simulink model "hdlcoder_led_blinking"  (R2026a)
settings: Solver=FixedStepDiscrete  StopTime=1
InitFcn:
  | Ts = 1e-3;
libraries: simulink x2, hdlsllib x2
settings Model: Creator=The MathWorks, Inc.  LastModifiedBy=The MathWorks, Inc.
settings OptimizationCC: ConditionallyExecuteInputs=off
settings DebuggingCC: AlgebraicLoopMsg=error  UnderspecifiedInitializationDetection=Classic  SingleTaskRateTransMsg=error  ParameterPrecisionLossMsg=none
settings HardwareCC: ProdHWDeviceType=ASIC/FPGA->ASIC/FPGA  ProdEqTarget=off

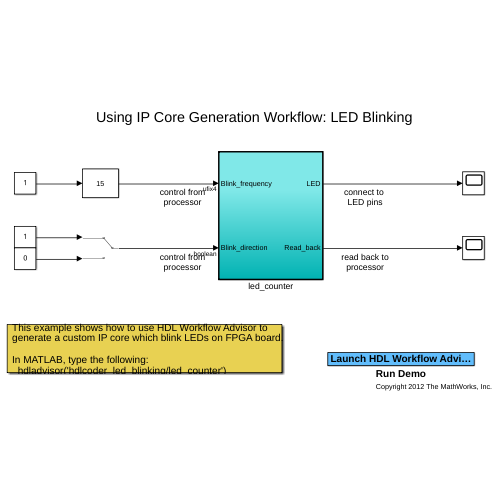
[thumbnail: Simulink's stored preview of the top-level diagram]
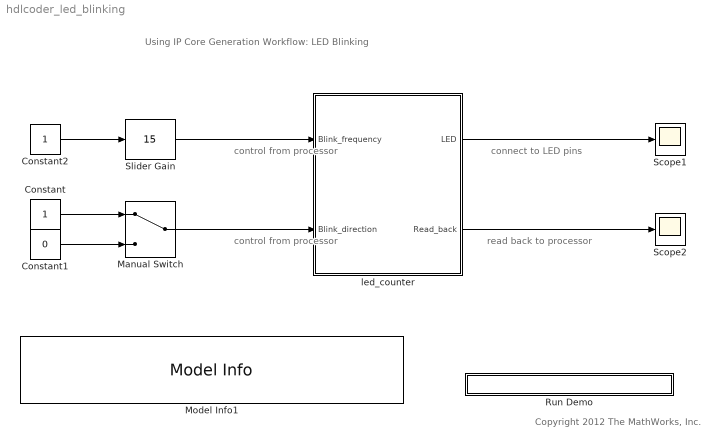
== system hdlcoder_led_blinking ==
  note: control from
      | processor
  note: Copyright 2012 The MathWorks, Inc.
  note: Using IP Core Generation Workflow: LED Blinking
  note: control from
      | processor
  note: connect to
      | LED pins
  note: read back to
      | processor
  Constant : Constant  OutDataTypeStr=boolean  SampleTime=Ts
  Constant1 : Constant  Value=0  OutDataTypeStr=boolean  SampleTime=Ts
  Constant2 : Constant  OutDataTypeStr=fixdt(0, 4, 0)  SampleTime=Ts
  Manual Switch : ManualSwitch
  Model Info1 : simulink/Model-Wide Utilities/Model Info  Frame=on  DisplayStringWithTags=|  HorizontalTextAlignment=Left  LeftAlignmentValue=0.02
      | This example shows how to use HDL Workflow Advisor to 
      | generate a custom IP core which blink LEDs on FPGA board.
      | 
      | In MATLAB, type the following:
      |   hdladvisor('hdlcoder_led_blinking/led_counter')
  Run Demo : Subsystem
      settings: OpenFcn=hdladvisor([bdroot, '/led_counter'])
      mask Display: disp('Launch HDL Workflow Advisor')
  Scope1 : Scope
  Scope2 : Scope
  Slider Gain : simulink/Math Operations/Slider Gain  gain=15  low=0  high=15
  led_counter : Subsystem  TreatAsAtomicUnit=on
  wires:
  Constant/1 -> Manual Switch/1
  Constant1/1 -> Manual Switch/2
  Manual Switch/1 -> led_counter/2(Blink_direction)
  Constant2/1 -> Slider Gain/1
  Slider Gain/1 -> led_counter/1(Blink_frequency)
  led_counter/2(Read_back) -> Scope2/1
  led_counter/1(LED) -> Scope1/1

== system hdlcoder_led_blinking/Run Demo ==

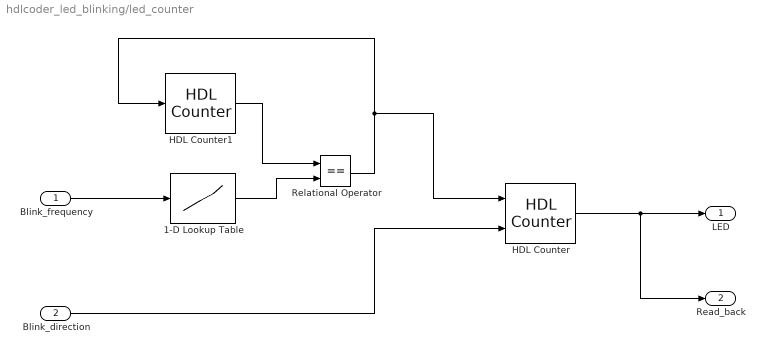
== system hdlcoder_led_blinking/led_counter ==
  Blink_frequency : Inport  OutDataTypeStr=fixdt(0, 4, 0)
  Blink_direction : Inport  Port=2  OutDataTypeStr=boolean
  1-D Lookup Table : Lookup_n-D  NumberOfTableDimensions=1  BreakpointsForDimension1=[0:15]  IndexSearchMethod=Evenly spaced points  Table=2.^[23:-1:8]  TableDataTypeStr=fixdt(0, 24, 0)  InterpMethod=Flat  DiagnosticForOutOfRangeInput=Error  OutDataTypeStr=fixdt(0, 24, 0)  RndMeth=Simplest
  HDL Counter : hdlsllib/Sources/HDL Counter  CountType=Free running  CountInit=0  CountStep=1  CountMax=100  CountFromType=Initial value  CountFrom=0  CountResetPort=off  CountLoadPort=off  CountEnbPort=on  CountDirPort=on  CountHitOutputPort=off  CountDataType=Unsigned  CountWordLen=8  CountFracLen=0  CountSampTime=1
  HDL Counter1 : hdlsllib/Sources/HDL Counter  CountType=Free running  CountInit=0  CountStep=1  CountMax=100  CountFromType=Initial value  CountFrom=0  CountResetPort=on  CountLoadPort=off  CountEnbPort=off  CountDirPort=off  CountHitOutputPort=off  CountDataType=Unsigned  CountWordLen=24  CountFracLen=0  CountSampTime=1
  Relational Operator : RelationalOperator  Operator===  OutDataTypeStr=boolean  InputSameDT=off
  LED : Outport  VectorParamsAs1DForOutWhenUnconnected=off
  Read_back : Outport  Port=2  VectorParamsAs1DForOutWhenUnconnected=off
  wires:
  HDL Counter/1 -> Read_back/1, LED/1
  HDL Counter1/1 -> Relational Operator/1
  Relational Operator/1 -> HDL Counter/1, HDL Counter1/1
  Blink_frequency/1 -> 1-D Lookup Table/1
  1-D Lookup Table/1 -> Relational Operator/2
  Blink_direction/1 -> HDL Counter/2
